simulink model "ref_basic_sources"  (R2026a)
settings: Solver=ode45  StopTime=3  FixedStep=1e-3  MaxStep=1e-2  RelTol=1e-10  AbsTol=1e-12
settings Model: Creator=djangovanderplas  LastModifiedBy=djangovanderplas
settings DataIOCC: OutputOption=SpecifiedOutputTimes  OutputTimes=0:1e-3:3

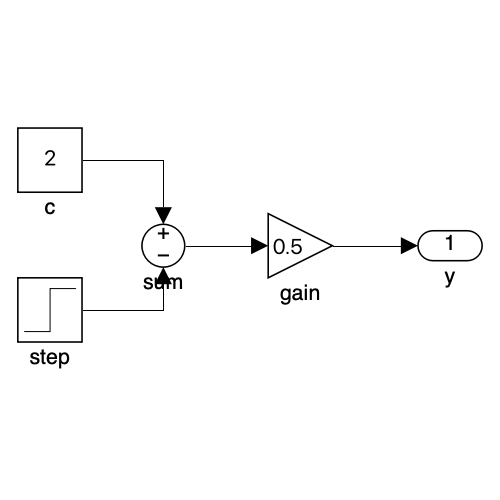
[thumbnail: Simulink's stored preview of the top-level diagram]
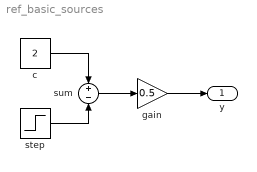
== system ref_basic_sources ==
  c : Constant  Value=2
  gain : Gain  Gain=0.5
  step : Step  FinalValue=3  SampleTime=0
  sum : Sum  Inputs=+-
  y : Outport
  wires:
  gain/1 -> y/1
  sum/1 -> gain/1
  step/1 -> sum/2
  c/1 -> sum/1
